simulink model "Dutch_Roll"  (R2022a)
settings: Solver=VariableStepAuto  StartTime=0.0  StopTime=2000  RelTol=1e-3
undefined symbols (not defined in the file): ADr, BDr, CDr, DDr
libraries: simulink_extras x2
settings Model: Creator=ks2-parmar  LastModifiedBy=ks2-parmar

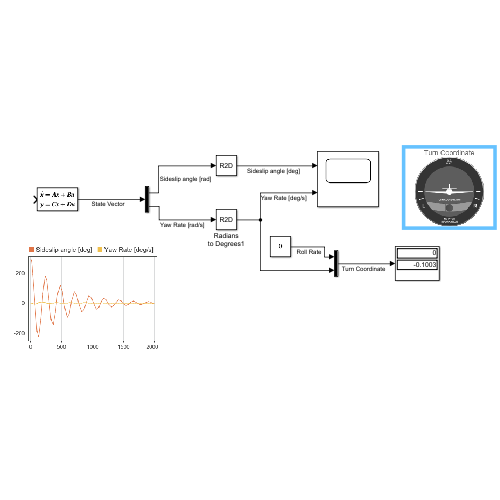
[thumbnail: Simulink's stored preview of the top-level diagram]
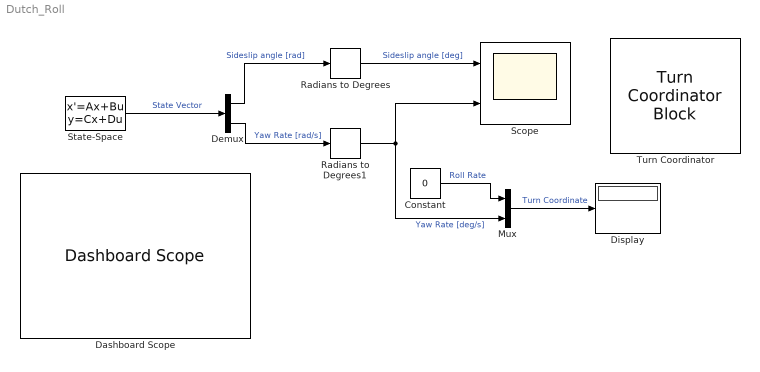
== system Dutch_Roll ==
  Constant : Constant  Value=0
  Dashboard Scope : DashboardScope
  Demux : Demux  Outputs=2
  Display : Display
  Mux : Mux  Inputs=2
  Radians to Degrees : simulink_extras/Transformations/Radians to Degrees
  Radians to Degrees1 : simulink_extras/Transformations/Radians to Degrees
  Scope : Scope  NumInputPorts=2
  State-Space : StateSpace  A=ADr  B=BDr  C=CDr  D=DDr  InitialCondition=[5;0]
  Turn Coordinator : TurnCoordinatorBlock
  wires:
  State-Space/1 -> Demux/1  "State Vector"
  Demux/1 -> Radians to Degrees/1  "Sideslip angle [rad]"
  Demux/2 -> Radians to Degrees1/1  "Yaw Rate [rad/s]"
  Constant/1 -> Mux/1  "Roll Rate"
  Radians to Degrees1/1 -> Scope/2, Mux/2  "Yaw Rate [deg/s]"
  Radians to Degrees/1 -> Scope/1  "Sideslip angle [deg]"
  Mux/1 -> Display/1  "Turn Coordinate"
